simulink model "offgrid_microgrid"  (R2024b)
settings: Solver=ode23tb  StartTime=0.0  StopTime=15  MaxStep=0.005  RelTol=1e-3
libraries: spsThreePhaseSeriesRLCLoadLib x2, spsThreePhaseDynamicLoadLib x1, spsThreePhaseVIMeasurementLib x1, spsSimplifiedSynchronousMachinepuUnitsLib x1, spsThreePhaseBreakerLib x1, sps_lib x1
settings Model: Creator=Md Sazzadur Rahman  LastModifiedBy=Md Sazzadur Rahman

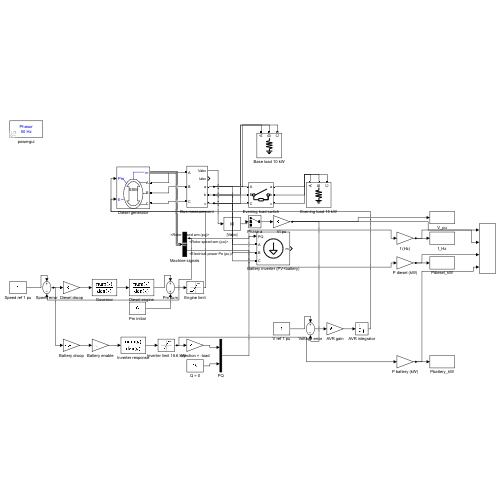
[thumbnail: Simulink's stored preview of the top-level diagram]
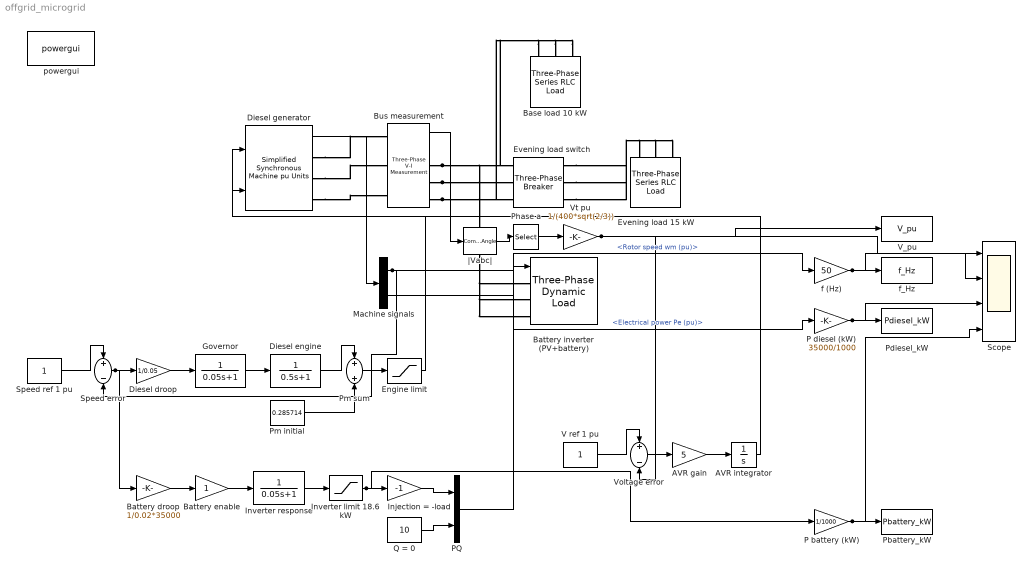
== system offgrid_microgrid ==
  AVR gain : Gain  Gain=5
  AVR integrator : Integrator  InitialCondition=1  LimitOutput=on  UpperSaturationLimit=2  LowerSaturationLimit=0.5
  Base load 10 kW : spsThreePhaseSeriesRLCLoadLib/Three-Phase Series RLC Load  LConnTagsString=A|B|C  Configuration=Y (grounded)  NominalVoltage=400  Vabc=[1e3 1e3 1e3]  Vabcp=[1e3 1e3 1e3]  NominalFrequency=50  UnbalancedPower=off  ActivePower=10000  InductivePower=0  CapacitivePower=0  Pabc=[10e3 9e3 11e3]  QLabc=[100 90 110]  QCabc=[100 90 110]  Pabcp=[10e3 9e3 11e3]  QLabcp=[100 90 110]  QCabcp=[100 90 110]  Measurements=None  LoadType=constant Z
  Battery droop : Gain  Gain=1/0.02*35000
  Battery enable : Gain
  Battery inverter (PV+battery) : spsThreePhaseDynamicLoadLib/Three-Phase Dynamic Load  NominalVoltage=[400 50]  ActiveReactivePowers=[0 10]  PositiveSequence=[1 0]  ExternalControl=on  NpNq=[0 0]  TimeConstants="[0  0  0  0]"  MinimumVoltage=0.7  Tfilter=1e-4  LoadFlowParameters=[4,0,0,0,0]
      settings: LibrarySourceBlock=|
      | sps_lib/Passives/Three-Phase
      | Dynamic Load
  Bus measurement : spsThreePhaseVIMeasurementLib/Three-Phase V-I Measurement  VoltageMeasurement=phase-to-ground  SetLabelV=off  LabelV=Vabc  Vpu=off  VpuLL=off  CurrentMeasurement=yes  SetLabelI=off  LabelI=Iabc  Ipu=off  Pbase=100e6  Vbase=500e3  OutputType=Complex  PhasorSimulation=on  PSBequivalent=0
  Diesel droop : Gain  Gain=1/0.05
  Diesel engine : TransferFcn  Numerator=1  Denominator=[0.5 1]
  Diesel generator : spsSimplifiedSynchronousMachinepuUnitsLib/Simplified Synchronous Machine pu Units  ConnectionType=3-wire Y  MechanicalLoad=Mechanical power Pm  MeasurementBus=off  NominalParameters=[35000 400 50]  Mechanical=[1 0 2]  InternalRL=[0.02 0.3]  InitialConditions="[ 0,0   0,0,0   0,0,0 ]"  IterativeDiscreteModel=Trapezoidal non iterative  TsBlock=-1  TsPowergui=0  LoadFlowParameters=[1,0,0,0,0]  Units=0  BusType=PV  Pref=0  Qref=0  Qmin=-inf  Qmax=+inf  PLF=0  QLF=0
      settings: LibrarySourceBlock=|
      | sps_lib/Electrical Machines/Simplified Synchronous
      | Machine pu Units
  Engine limit : Saturate  UpperLimit=1.1  LowerLimit=0
  Evening load 15 kW : spsThreePhaseSeriesRLCLoadLib/Three-Phase Series RLC Load  LConnTagsString=A|B|C  Configuration=Y (grounded)  NominalVoltage=400  Vabc=[1e3 1e3 1e3]  Vabcp=[1e3 1e3 1e3]  NominalFrequency=50  UnbalancedPower=off  ActivePower=15000  InductivePower=0  CapacitivePower=0  Pabc=[10e3 9e3 11e3]  QLabc=[100 90 110]  QCabc=[100 90 110]  Pabcp=[10e3 9e3 11e3]  QLabcp=[100 90 110]  QCabcp=[100 90 110]  Measurements=None  LoadType=constant Z
  Evening load switch : spsThreePhaseBreakerLib/Three-Phase Breaker  InitialState=open  SwitchA=on  SwitchB=on  SwitchC=on  SwitchTimes=[5]  External=off  BreakerResistance=0.01  SnubberResistance=1e6  SnubberCapacitance=inf  Measurements=None
  Governor : TransferFcn  Numerator=1  Denominator=[0.05 1]
  Injection = -load : Gain  Gain=-1
  Inverter limit 18.6 kW : Saturate  UpperLimit=18600  LowerLimit=-18600
  Inverter response : TransferFcn  Numerator=1  Denominator=[0.05 1]
  Machine signals : BusSelector  OutputSignals=Rotor speed wm (pu),Electrical power Pe (pu)
  P battery (kW) : Gain  Gain=1/1000
  P diesel (kW) : Gain  Gain=35000/1000
  PQ : Mux  Inputs=2
  Pbattery_kW : ToWorkspace  VariableName=Pbattery_kW  SaveFormat=Structure With Time  SampleTime=-1
  Pdiesel_kW : ToWorkspace  VariableName=Pdiesel_kW  SaveFormat=Structure With Time  SampleTime=-1
  Phase a : Selector  InputPortWidth=3  IndexOptions=Index vector (dialog)  Indices=1  OutputSizes=1
  Pm initial : Constant  Value=0.285714
  Pm sum : Sum
  Q = 0 : Constant  Value=10
  Scope : Scope  NumInputPorts=4
  Speed error : Sum  Inputs=+-
  Speed ref 1 pu : Constant
  V ref 1 pu : Constant
  V_pu : ToWorkspace  VariableName=V_pu  SaveFormat=Structure With Time  SampleTime=-1
  Voltage error : Sum  Inputs=+-
  Vt pu : Gain  Gain=1/(400*sqrt(2/3))
  f (Hz) : Gain  Gain=50
  f_Hz : ToWorkspace  VariableName=f_Hz  SaveFormat=Structure With Time  SampleTime=-1
  powergui : sps_lib/powergui  Priority=1  SimulationMode=Phasor  SampleTime=50e-6  frequency=50  Iterations=50  frequencyindice=50  Pbase=100e6  ErrMax=1e-4  UnitsV=kV  UnitsW=MW  buscounter=0  FunctionMessages=off  echomessages=off  EnableUseOfTLC=off  CurrentSourceSwitches=off  DisableSnubberDevices=off  DisableRonSwitches=off  DisableVfSwitches=off  DisplayEquations=off  AutomaticDiscreteSolvers=off  SolverType=Tustin/Backward Euler (TBE)  Interpol=off  ExternalGateDelay=off  methode=off  Ts=100  x0status=blocks  SPID=on  SwTol=0  HookPort=off  NonlinearTolerance=1e-4  nMaxIteration=100  ContinueOnMaxIteration=off  RestoreLinks=warning  ResistiveCurrentMeasurement=off  Frange=50  Ylog=off  Xlog=on  ShowGrid=off  save=off  variable=ZData  structure=0  ZoomFFT=off  StartTime=0.0  cycles=1  DisplayStyle=1  fundamental=60  FreqAxis=off  MaxFrequency=50  frequencyindicesteady=50  RmsSteady=1  display=off
  |Vabc| : ComplexToMagnitudeAngle  Output=Magnitude
  wires:
  Diesel generator/1 -> Machine signals/1
  Machine signals/1 -> Speed error/2, f (Hz)/1  "<Rotor speed wm (pu)>"
  Speed ref 1 pu/1 -> Speed error/1
  Speed error/1 -> Diesel droop/1, Battery droop/1
  Diesel droop/1 -> Governor/1
  Governor/1 -> Diesel engine/1
  Diesel engine/1 -> Pm sum/1
  Pm initial/1 -> Pm sum/2
  Pm sum/1 -> Engine limit/1
  Engine limit/1 -> Diesel generator/1
  Bus measurement/1 -> |Vabc|/1
  |Vabc|/1 -> Phase a/1
  Phase a/1 -> Vt pu/1
  V ref 1 pu/1 -> Voltage error/1
  Vt pu/1 -> Voltage error/2, V_pu/1, Scope/2
  Voltage error/1 -> AVR gain/1
  AVR gain/1 -> AVR integrator/1
  AVR integrator/1 -> Diesel generator/2
  Battery droop/1 -> Battery enable/1
  Battery enable/1 -> Inverter response/1
  Inverter response/1 -> Inverter limit 18.6 kW/1
  Inverter limit 18.6 kW/1 -> Injection = -load/1, P battery (kW)/1
  Injection = -load/1 -> PQ/1
  Q = 0/1 -> PQ/2
  PQ/1 -> Battery inverter (PV+battery)/1
  Machine signals/2 -> P diesel (kW)/1  "<Electrical power Pe (pu)>"
  f (Hz)/1 -> f_Hz/1, Scope/1
  P diesel (kW)/1 -> Pdiesel_kW/1, Scope/3
  P battery (kW)/1 -> Pbattery_kW/1, Scope/4
  connections:
  Diesel generator/RConn1 -- Bus measurement/LConn1
  Base load 10 kW/LConn1 -- Bus measurement/RConn1 -- Evening load switch/LConn1 -- Battery inverter (PV+battery)/LConn1
  Evening load switch/RConn1 -- Evening load 15 kW/LConn1
  Diesel generator/RConn2 -- Bus measurement/LConn2
  Base load 10 kW/LConn2 -- Bus measurement/RConn2 -- Evening load switch/LConn2 -- Battery inverter (PV+battery)/LConn2
  Evening load switch/RConn2 -- Evening load 15 kW/LConn2
  Diesel generator/RConn3 -- Bus measurement/LConn3
  Base load 10 kW/LConn3 -- Bus measurement/RConn3 -- Evening load switch/LConn3 -- Battery inverter (PV+battery)/LConn3
  Evening load switch/RConn3 -- Evening load 15 kW/LConn3
